simulink model "adrc_main"  (R2025b)
settings: Solver=VariableStepAuto  StartTime=0.0  StopTime=20  RelTol=1e-4
values from neighbouring files (symbols this model uses):
  Alloc = [ kf,     kf,     kf,     kf ... (first row only)    [quad_params.m]
  Area = 2*L*Width    (= 0.072)    [quad_params.m]
  g = 9.81    [quad_params.m]
  h = [0 ... (first row only)    [Madgwick.m]    (also in quad_params.m = 0.2; umich_learning.m = x(:,1))
  h0 = Ts    (= 0.001)    [quad_params.m]
  inertia_mx = [Ixx; Iyy; Izz;]    [quad_params.m]
  init_h = 0.03    [quad_params.m]
  K_alloc = Alloc \ diag([W, 1, 1, 1])    [quad_params.m]
  max_rad_s_2 = max_rad_s ^ 2    (= 4279618.17072)    [quad_params.m]
  max_thrust = max_rad_s_2 * kf * 4    (= 26.9016798211)    [quad_params.m]
  r0_position = 1    [quad_params.m]
  rho_air = 1.225    [quad_params.m]
  rho_water = 1000    [quad_params.m]
  Trot = 0.01    [quad_params.m]
  Ts = 0.001    [get_noise.m]    (also in quad_params.m; test.m = 0.002)
  W = 0.7 + 4*m_prop    (= 0.74)    [quad_params.m]
undefined symbols (not defined in the file or in its folder): adrc
libraries: simulink x4, aerolibwind2 x1
settings Model: PacingRate=0.400000  Creator=David  LastModifiedBy=David

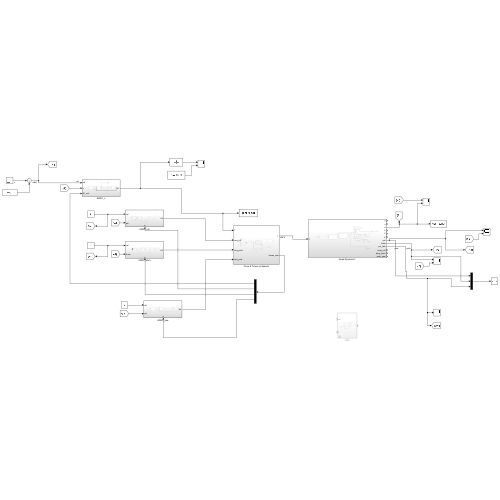
[thumbnail: Simulink's stored preview of the top-level diagram]
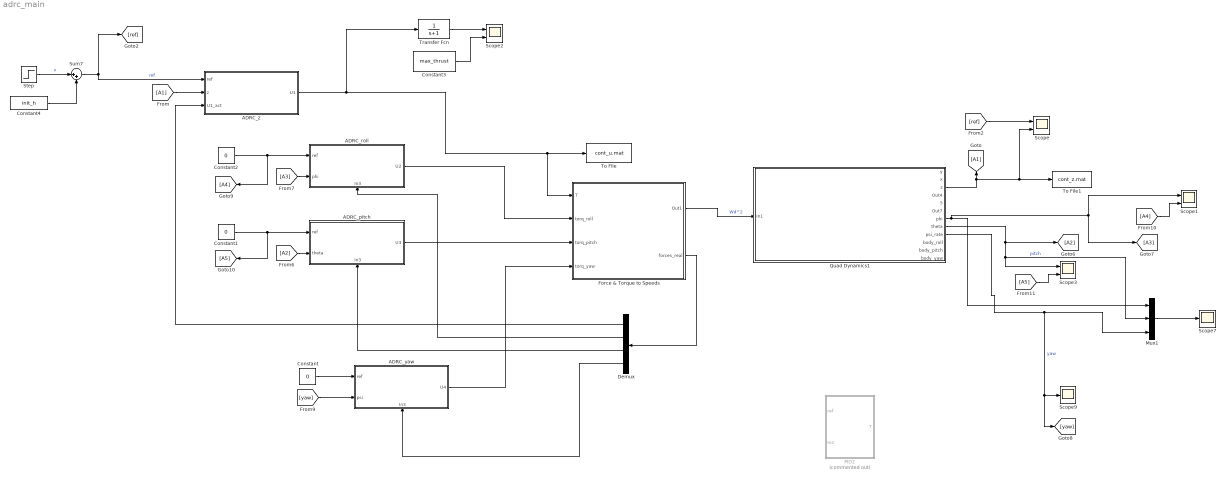
== system adrc_main ==
  ADRC_pitch : Subsystem
      settings: PortSchema="{\"entries\":[{\"content\":{\"sides\":[{\"content\":{\"connectorIds\":[\"In1\",\"In2\"]},\"type\":\"ConnectorPlacement.EquallySpacedRectSide\",\"uuid\":\"6cc80560-d5fb-4d70-bab2-c51ed037dc75\"},{\"content\":{\"connectorIds\":[\"Out1\"],\"side\":\"RIGHT\"},\"type\":\"ConnectorPlacement.EquallySpacedRectSide\",\"uuid\":\"11bda7cd-3ac7-47c0-848b-d0ab204a3c3d\"},{\"content\":{\"side\":\"TOP\"},\"type\":\"ConnectorPlacement.EquallySpacedRectSide\",\"uuid\":\"2a4fd4ae-6a0e-48eb-9f11-b11d2041070f\"},{\"content\":{\"connectorIds\":[\"In3\"],\"side\":\"BOTTOM\"},\"type\":\"ConnectorPlacement.EquallySpacedRectSide\",\"uuid\":\"f4a2dede-c3a4-45a0-96a3-5f68fdbf4ab0\"}]},\"type\":\"ConnectorPlacement.EquallySpacedConnector\",\"uuid\":\"bf44a222-f2d1-4d7f-8b8f-a2aef4aa21c8\"}],\"packageUris\":[\"http://schema.mathworks.com/mf0/Connector/R2020b\"],\"version\":\"1.0\"}"
  ADRC_roll : Subsystem
      settings: PortSchema="{\"entries\":[{\"content\":{\"sides\":[{\"content\":{\"connectorIds\":[\"In1\",\"In2\"]},\"type\":\"ConnectorPlacement.EquallySpacedRectSide\",\"uuid\":\"6cc80560-d5fb-4d70-bab2-c51ed037dc75\"},{\"content\":{\"connectorIds\":[\"Out1\"],\"side\":\"RIGHT\"},\"type\":\"ConnectorPlacement.EquallySpacedRectSide\",\"uuid\":\"11bda7cd-3ac7-47c0-848b-d0ab204a3c3d\"},{\"content\":{\"side\":\"TOP\"},\"type\":\"ConnectorPlacement.EquallySpacedRectSide\",\"uuid\":\"2a4fd4ae-6a0e-48eb-9f11-b11d2041070f\"},{\"content\":{\"connectorIds\":[\"In3\"],\"side\":\"BOTTOM\"},\"type\":\"ConnectorPlacement.EquallySpacedRectSide\",\"uuid\":\"852e14b7-d2e0-4511-9e4e-b55cc1d4afdd\"}]},\"type\":\"ConnectorPlacement.EquallySpacedConnector\",\"uuid\":\"bf44a222-f2d1-4d7f-8b8f-a2aef4aa21c8\"}],\"packageUris\":[\"http://schema.mathworks.com/mf0/Connector/R2020b\"],\"version\":\"1.0\"}"
  ADRC_yaw : Subsystem
      settings: PortSchema="{\"entries\":[{\"content\":{\"sides\":[{\"content\":{\"connectorIds\":[\"In1\",\"In2\"]},\"type\":\"ConnectorPlacement.EquallySpacedRectSide\",\"uuid\":\"6cc80560-d5fb-4d70-bab2-c51ed037dc75\"},{\"content\":{\"connectorIds\":[\"Out1\"],\"side\":\"RIGHT\"},\"type\":\"ConnectorPlacement.EquallySpacedRectSide\",\"uuid\":\"11bda7cd-3ac7-47c0-848b-d0ab204a3c3d\"},{\"content\":{\"side\":\"TOP\"},\"type\":\"ConnectorPlacement.EquallySpacedRectSide\",\"uuid\":\"2a4fd4ae-6a0e-48eb-9f11-b11d2041070f\"},{\"content\":{\"connectorIds\":[\"In3\"],\"side\":\"BOTTOM\"},\"type\":\"ConnectorPlacement.EquallySpacedRectSide\",\"uuid\":\"76ba5801-5866-4633-be25-22afc3afb05e\"}]},\"type\":\"ConnectorPlacement.EquallySpacedConnector\",\"uuid\":\"bf44a222-f2d1-4d7f-8b8f-a2aef4aa21c8\"}],\"packageUris\":[\"http://schema.mathworks.com/mf0/Connector/R2020b\"],\"version\":\"1.0\"}"
  ADRC_z : Subsystem
  Constant : Constant  Value=0
  Constant1 : Constant  Value=0
  Constant2 : Constant  Value=0
  Constant3 : Constant  Value=max_thrust
  Constant4 : Constant  Value=init_h
  Demux : Demux
  Force & Torque to Speeds : Subsystem
  Mux1 : Mux  Inputs=3
  PID2 : Subsystem  Commented=on
  Quad Dynamics1 : Subsystem
  Scope{,1..3} (4 alike) : Scope  NumInputPorts=2
      Scope settings: ActiveDisplayYMinimum=-0.13072157560972555  ActiveDisplayYMaximum=1.1764941804875302  DataLoggingVariableName=ScopeData2
      Scope1 settings: ActiveDisplayYMinimum=-0.066210271925645478  ActiveDisplayYMaximum=0.59589244733080937
      Scope2 settings: ActiveDisplayYMinimum=-1  ActiveDisplayYMaximum=1  DataLoggingVariableName=ScopeData5
      Scope3 settings: ActiveDisplayYMinimum=-0.25349599567622344  ActiveDisplayYMaximum=0.40002228208849239
  Scope7 : Scope
      settings: ActiveDisplayYMinimum=-0.926750348726782  ActiveDisplayYMaximum=1.337695858172476  DataLoggingVariableName=ScopeData16
  Scope9 : Scope
      settings: ActiveDisplayYMinimum=-327.86369595183078  ActiveDisplayYMaximum=1369.6610229277119  DataLoggingVariableName=ScopeData15
  Step : Step  Time=2  SampleTime=0
  Sum7 : Sum  Inputs=|++
  To File : ToFile  Filename=cont_u.mat  SaveFormat=Timeseries
  To File1 : ToFile  Filename=cont_z.mat  SaveFormat=Timeseries
  Transfer Fcn : TransferFcn  Denominator=[1 1]
  wires:
  Quad Dynamics1/3(z) -> To File1/1, Scope/2, [A1]
  [A1] -> ADRC_z/2(z)
  Constant2/1 -> ADRC_roll/1(ref), [A4]
  Constant1/1 -> [A5], ADRC_pitch/1(ref)
  [A2] -> ADRC_pitch/2(theta)
  [A3] -> ADRC_roll/2(phi)
  [yaw] -> ADRC_yaw/2(psi)
  Force & Torque to Speeds/1(Out1) -> Quad Dynamics1/1(In1)  "Wd^2"
  ADRC_z/1(U1) -> Transfer Fcn/1, To File/1, Force & Torque to Speeds/1(T)
  [A4] -> Scope1/2
  [A5] -> Scope3/2
  Quad Dynamics1/9(psi_rate) -> Mux1/3, Scope9/1, [yaw]  "yaw"
  Quad Dynamics1/8(theta) -> [A2], Mux1/2, Scope3/1  "pitch"
  Constant/1 -> ADRC_yaw/1(ref)
  Quad Dynamics1/7(phi) -> Mux1/1, Scope1/1, [A3]
  Force & Torque to Speeds/2(forces_real) -> Demux/1
  Demux/1 -> ADRC_z/3(U1_act)
  Demux/3 -> ADRC_pitch/3(In3)
  Demux/4 -> ADRC_yaw/3(In3)
  Demux/2 -> ADRC_roll/3(In3)
  [ref] -> Scope/1
  Sum7/1 -> [ref], ADRC_z/1(ref)  "ref"
  Step/1 -> Sum7/1  "v"
  Constant4/1 -> Sum7/2
  Mux1/1 -> Scope7/1
  Constant3/1 -> Scope2/2
  Transfer Fcn/1 -> Scope2/1
  ADRC_pitch/1(U3) -> Force & Torque to Speeds/3(torq_pitch)
  ADRC_roll/1(U2) -> Force & Torque to Speeds/2(torq_roll)
  ADRC_yaw/1(U4) -> Force & Torque to Speeds/4(torq_yaw)

== system adrc_main/ADRC_pitch ==
  ref : Inport
  theta : Inport  Port=2
  In3 : Inport  Port=3
  Bus Selector1 : BusSelector  Commented=on  OutputSignals=x3,x1
  LADRC1 : Subsystem
  LESO : Subsystem
  Scope : Scope  NumInputPorts=2
      settings: ActiveDisplayYMinimum=-0.19035360050017919  ActiveDisplayYMaximum=0.29946548587767807  DataLoggingVariableName=ScopeData3
  Scope1 : Scope  NumInputPorts=2
      settings: ActiveDisplayYMinimum=-1.7064424027385405  ActiveDisplayYMaximum=1.5214383476696569  DataLoggingVariableName=ScopeData9
  Scope6 : Scope  Commented=on
      settings: ActiveDisplayYMinimum=-1.7735639903680922  ActiveDisplayYMaximum=2.4901305931130953  DataLoggingVariableName=ScopeData11
  Scope7 : Scope  Commented=on  NumInputPorts=2
      settings: ActiveDisplayYMinimum=-10.826635982413356  ActiveDisplayYMaximum=4.5963077407770285  DataLoggingVariableName=ScopeData7
  Transfer Fcn : TransferFcn  Commented=on  Denominator=[0.8 1]
  Transfer Fcn1 : TransferFcn  Numerator=[1 0]  Denominator=[Ts 1]
  U3 : Outport
  wires:
  Transfer Fcn/1 -> Scope7/2
  ref/1 -> LADRC1/1(ref), Scope/1, Transfer Fcn1/1, Scope/2
  LESO/1(z_hat) -> LADRC1/2(x_hat), Bus Selector1/1
  theta/1 -> LESO/1(theta)
  Bus Selector1/1 -> Transfer Fcn/1, Scope7/1  "<x3>"
  Bus Selector1/2 -> Scope6/1  "<x1>"
  LADRC1/1(U3) -> Scope1/2, U3/1
  Transfer Fcn1/1 -> LADRC1/3(ref_dot)
  In3/1 -> Scope1/1, LESO/2(U3)

== system adrc_main/ADRC_roll ==
  ref : Inport
  phi : Inport  Port=2
  In3 : Inport  Port=3
  Bus Selector1 : BusSelector  Commented=on  OutputSignals=x3,x1
  LADRC1 : Subsystem
  LESO1 : Subsystem
  Scope : Scope  NumInputPorts=2
      settings: ActiveDisplayYMinimum=-0.25662655483048824  ActiveDisplayYMaximum=0.1660137932117976  DataLoggingVariableName=ScopeData25
  Scope1 : Scope  NumInputPorts=2
      settings: ActiveDisplayYMinimum=-1.3986509021572997  ActiveDisplayYMaximum=1.4330939530069289  DataLoggingVariableName=ScopeData14
  Scope6 : Scope  Commented=on
      settings: ActiveDisplayYMinimum=-1.7735639903680922  ActiveDisplayYMaximum=2.4901305931130953  DataLoggingVariableName=ScopeData11
  Scope7 : Scope  Commented=on  NumInputPorts=2
      settings: ActiveDisplayYMinimum=-10.826635982413356  ActiveDisplayYMaximum=4.5963077407770285  DataLoggingVariableName=ScopeData7
  Transfer Fcn : TransferFcn  Commented=on  Denominator=[0.8 1]
  Transfer Fcn1 : TransferFcn  Numerator=[1 0]  Denominator=[Ts 1]
  U2 : Outport
  wires:
  Bus Selector1/2 -> Scope6/1  "<x1>"
  Bus Selector1/1 -> Scope7/1, Transfer Fcn/1  "<x3>"
  phi/1 -> LESO1/1(phi)
  LESO1/1(z_hat) -> LADRC1/2(x_hat)
  Transfer Fcn/1 -> Scope7/2
  Transfer Fcn1/1 -> LADRC1/3(ref_dot)
  ref/1 -> Scope/1, LADRC1/1(ref), Transfer Fcn1/1, Scope/2
  LADRC1/1(U2) -> Scope1/2, U2/1
  In3/1 -> Scope1/1, LESO1/2(U2)

== system adrc_main/ADRC_yaw ==
  ref : Inport
  psi : Inport  Port=2
  In3 : Inport  Port=3
  LADRC1 : Subsystem
  LESO1 : Subsystem
  TD1 : Subsystem
  U4 : Outport
  wires:
  TD1/1(ref) -> LADRC1/1(ref)
  LESO1/1(x_hat) -> LADRC1/2(x_hat)
  psi/1 -> LESO1/1(psi)
  TD1/2(dref) -> LADRC1/3(ref_dot)
  ref/1 -> TD1/1(v)
  In3/1 -> LESO1/2(U4)  "U4_real"
  LADRC1/1(U4) -> U4/1

== system adrc_main/ADRC_z ==
  ref : Inport
  z : Inport  Port=2
  U1_act : Inport  Port=3
  Gain1 : Gain  Gain=1/W
  LADRC1 : Subsystem
  LESO1 : Subsystem
  Scope1 : Scope  NumInputPorts=2
      settings: ActiveDisplayYMinimum=-37.94825498232003  ActiveDisplayYMaximum=51.771622737675379  DataLoggingVariableName=ScopeData21
  TD1 : Subsystem
  U1 : Outport
  wires:
  ref/1 -> TD1/1(v)
  TD1/2(dref) -> LADRC1/3(ref_dot)
  LADRC1/1(U1) -> Scope1/1, Gain1/1
  z/1 -> LESO1/1(z)
  LESO1/1(z_hat) -> LADRC1/2(x_hat)
  TD1/1(ref) -> LADRC1/1(ref)
  Gain1/1 -> U1/1
  U1_act/1 -> LESO1/2(U1), Scope1/2

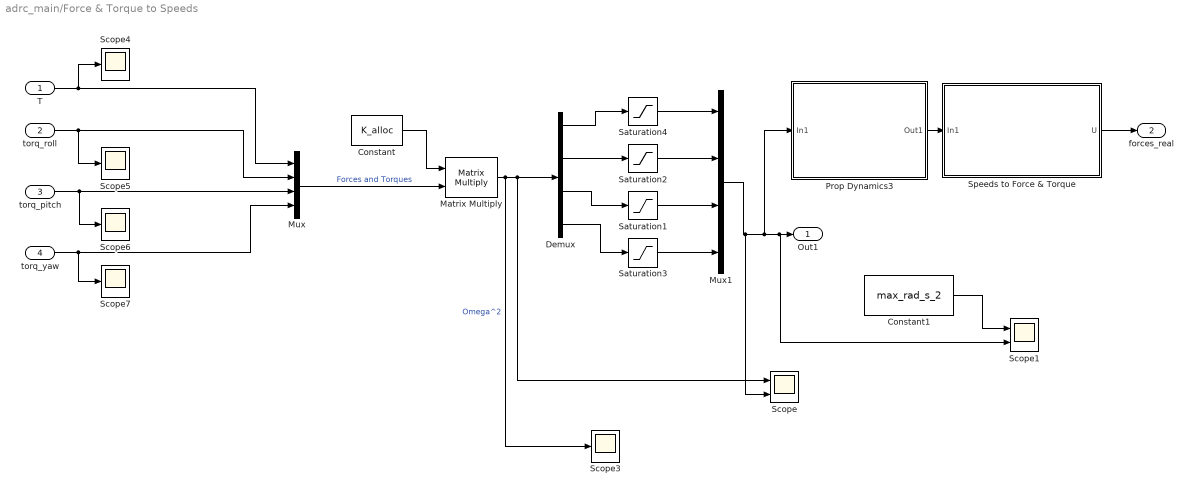
== system adrc_main/Force & Torque to Speeds ==
  T : Inport
  torq_roll : Inport  Port=2
  torq_pitch : Inport  Port=3
  torq_yaw : Inport  Port=4
  Constant : Constant  Value=K_alloc
  Constant1 : Constant  Value=max_rad_s_2
  Demux : Demux
  Matrix Multiply : Product  Multiplication=Matrix(*)
  Mux : Mux
  Mux1 : Mux
  Prop Dynamics3 : Subsystem
  Saturation{1..4} (4 alike) : Saturate  UpperLimit=max_rad_s_2  LowerLimit=0
  Scope : Scope  NumInputPorts=2
      settings: ActiveDisplayYMinimum=-1.1832105851156231E+7  ActiveDisplayYMaximum=1.5311490525694614E+7  DataLoggingVariableName=ScopeData11
  Scope1 : Scope  NumInputPorts=2
      settings: ActiveDisplayYMinimum=-845917.28935251338  ActiveDisplayYMaximum=5.3988813885811847E+6  DataLoggingVariableName=ScopeData25
  Scope{3..7} (5 alike) : Scope
      Scope3 settings: ActiveDisplayYMinimum=-1.1545612320423638E+7  ActiveDisplayYMaximum=1.430543184800574E+7  DataLoggingVariableName=ScopeData24
      Scope4 settings: ActiveDisplayYMinimum=-18.530778781079604  ActiveDisplayYMaximum=17.95290772841328  DataLoggingVariableName=ScopeData27
      Scope5 settings: ActiveDisplayYMinimum=-27.408261850577894  ActiveDisplayYMaximum=37.37109305567089  DataLoggingVariableName=ScopeData28
      Scope6 settings: ActiveDisplayYMinimum=-27.408261850577894  ActiveDisplayYMaximum=37.37109305567089  DataLoggingVariableName=ScopeData29
      Scope7 settings: ActiveDisplayYMinimum=-27.408261850577894  ActiveDisplayYMaximum=37.37109305567089  DataLoggingVariableName=ScopeData30
  Speeds to Force & Torque : Subsystem
  Out1 : Outport
  forces_real : Outport  Port=2
  wires:
  Matrix Multiply/1 -> Scope3/1, Scope/1, Demux/1  "Omega^2"
  torq_yaw/1 -> Mux/4, Scope7/1
  torq_pitch/1 -> Mux/3, Scope6/1
  torq_roll/1 -> Mux/2, Scope5/1
  T/1 -> Mux/1, Scope4/1
  Constant/1 -> Matrix Multiply/1
  Mux/1 -> Matrix Multiply/2  "Forces and Torques"
  Saturation3/1 -> Mux1/4
  Demux/4 -> Saturation3/1
  Demux/2 -> Saturation2/1
  Demux/1 -> Saturation4/1
  Demux/3 -> Saturation1/1
  Saturation2/1 -> Mux1/2
  Saturation4/1 -> Mux1/1
  Saturation1/1 -> Mux1/3
  Mux1/1 -> Scope/2, Scope1/2, Out1/1, Prop Dynamics3/1(In1)
  Speeds to Force & Torque/1(U) -> forces_real/1
  Prop Dynamics3/1(Out1) -> Speeds to Force & Torque/1(In1)
  Constant1/1 -> Scope1/1

== system adrc_main/PID2 ==
  ref : Inport
  In2 : Inport  Port=2
  Gain : Gain  Gain=90
  Gain1 : Gain  Gain=20
  Gain2 : Gain  Gain=30
  Scope : Scope  NumInputPorts=3
      settings: ActiveDisplayYMinimum=-207.05131739453731  ActiveDisplayYMaximum=124.29017503107066  DataLoggingVariableName=ScopeData6
  Sum : Sum  Inputs=|+-
  Sum1 : Sum  Inputs=|+++
  Transfer Fcn : TransferFcn  Numerator=[1 0]  Denominator=[0.01 1]
  Transfer Fcn1 : TransferFcn  Denominator=[1 0]
  T : Outport
  wires:
  In2/1 -> Sum/2
  ref/1 -> Sum/1
  Sum/1 -> Gain2/1, Gain/1, Gain1/1
  Gain1/1 -> Transfer Fcn/1
  Gain2/1 -> Transfer Fcn1/1
  Gain/1 -> Scope/2, Sum1/1  "P"
  Transfer Fcn1/1 -> Sum1/3, Scope/1  "I"
  Transfer Fcn/1 -> Scope/3, Sum1/2  "D"
  Sum1/1 -> T/1

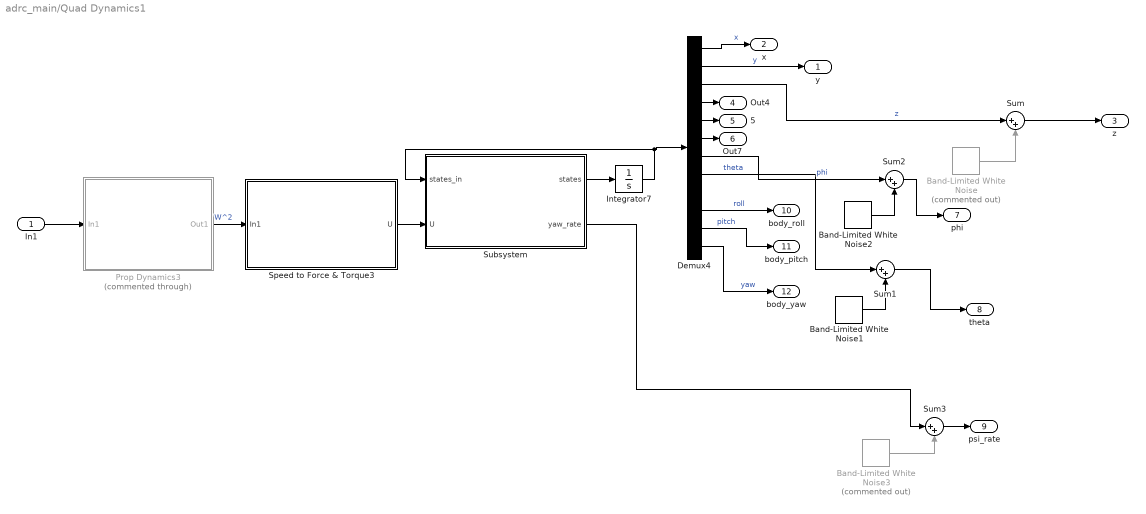
== system adrc_main/Quad Dynamics1 ==
  In1 : Inport
  Band-Limited White Noise : simulink/Sources/Band-Limited White Noise  Commented=on  Cov=[2.6540e-06]  Ts=0.02  seed=[23341]
  Band-Limited White Noise1 : simulink/Sources/Band-Limited White Noise  Cov=[2e-6]  Ts=0.001  seed=[23342]
  Band-Limited White Noise2 : simulink/Sources/Band-Limited White Noise  Cov=[2e-6]  Ts=0.001  seed=[23341]
  Band-Limited White Noise3 : simulink/Sources/Band-Limited White Noise  Commented=on  Cov=[0.0021446]  Ts=0.001  seed=[23343]
  Demux4 : Demux  Outputs=12
  Integrator7 : Integrator  InitialCondition=zeros(12,1)
  Prop Dynamics3 : Subsystem  Commented=through
  Speed to Force & Torque3 : Subsystem
  Subsystem : Subsystem
  Sum{,1..3} (4 alike) : Sum  Inputs=|++
  y : Outport
  x : Outport  Port=2
  z : Outport  Port=3
  Out4 : Outport  Port=4
  5 : Outport  Port=5
  Out7 : Outport  Port=6
  phi : Outport  Port=7
  theta : Outport  Port=8
  psi_rate : Outport  Port=9
  body_roll : Outport  Port=10
  body_pitch : Outport  Port=11
  body_yaw : Outport  Port=12
  wires:
  Demux4/2 -> y/1  "y"
  Prop Dynamics3/1(Out1) -> Speed to Force & Torque3/1(In1)  "W^2"
  Demux4/1 -> x/1  "x"
  Subsystem/1(states) -> Integrator7/1
  Speed to Force & Torque3/1(U) -> Subsystem/2(U)
  Integrator7/1 -> Demux4/1, Subsystem/1(states_in)
  Demux4/10 -> body_roll/1  "roll"
  Demux4/7 -> Sum2/1  "phi"
  Demux4/3 -> Sum/1  "z"
  Demux4/8 -> Sum1/1  "theta"
  Demux4/11 -> body_pitch/1  "pitch"
  Demux4/12 -> body_yaw/1  "yaw"
  Demux4/6 -> Out7/1
  Demux4/5 -> 5/1
  Demux4/4 -> Out4/1
  In1/1 -> Prop Dynamics3/1(In1)
  Subsystem/2(yaw_rate) -> Sum3/1
  Sum/1 -> z/1
  Band-Limited White Noise/1 -> Sum/2
  Band-Limited White Noise1/1 -> Sum1/2
  Sum1/1 -> theta/1
  Band-Limited White Noise2/1 -> Sum2/2
  Sum2/1 -> phi/1
  Band-Limited White Noise3/1 -> Sum3/2
  Sum3/1 -> psi_rate/1

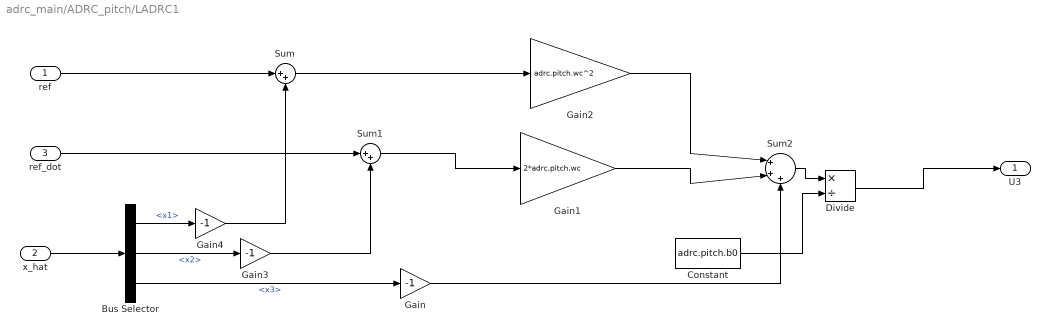
== system adrc_main/ADRC_pitch/LADRC1 ==
  ref : Inport
  x_hat : Inport  Port=2
  ref_dot : Inport  Port=3
  Bus Selector : BusSelector  OutputSignals=x1,x2,x3
  Constant : Constant  Value=adrc.pitch.b0
  Divide : Product  Inputs=*/
  Gain : Gain  Gain=-1
  Gain1 : Gain  Gain=2*adrc.pitch.wc
  Gain2 : Gain  Gain=adrc.pitch.wc^2
  Gain3 : Gain  Gain=-1
  Gain4 : Gain  Gain=-1
  Sum : Sum  Inputs=|++
  Sum1 : Sum  Inputs=|++
  Sum2 : Sum  Inputs=|+++
  U3 : Outport
  wires:
  ref_dot/1 -> Sum1/1
  x_hat/1 -> Bus Selector/1
  Bus Selector/3 -> Gain/1  "<x3>"
  Gain2/1 -> Sum2/1
  Gain/1 -> Sum2/3
  Gain1/1 -> Sum2/2
  Bus Selector/1 -> Gain4/1  "<x1>"
  Bus Selector/2 -> Gain3/1  "<x2>"
  Gain4/1 -> Sum/2
  Gain3/1 -> Sum1/2
  Sum1/1 -> Gain1/1
  Divide/1 -> U3/1
  ref/1 -> Sum/1
  Sum/1 -> Gain2/1
  Sum2/1 -> Divide/1
  Constant/1 -> Divide/2

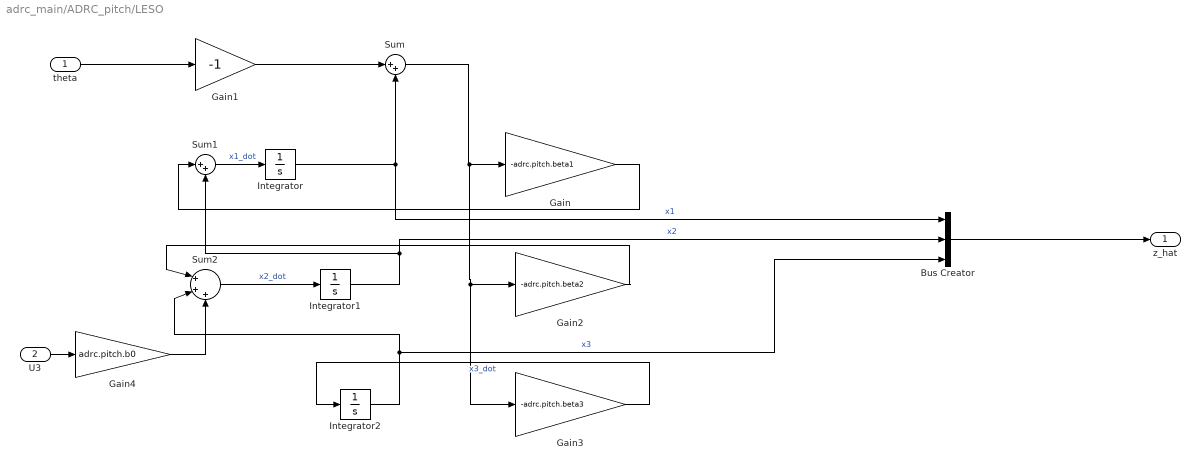
== system adrc_main/ADRC_pitch/LESO ==
  theta : Inport
  U3 : Inport  Port=2
  Bus Creator : BusCreator  Inputs=3
  Gain : Gain  Gain=-adrc.pitch.beta1
  Gain1 : Gain  Gain=-1
  Gain2 : Gain  Gain=-adrc.pitch.beta2
  Gain3 : Gain  Gain=-adrc.pitch.beta3
  Gain4 : Gain  Gain=adrc.pitch.b0
  Integrator : Integrator
  Integrator1 : Integrator
  Integrator2 : Integrator
  Sum : Sum  Inputs=|++
  Sum1 : Sum  Inputs=|++
  Sum2 : Sum  Inputs=|+++
  z_hat : Outport
  wires:
  theta/1 -> Gain1/1
  Gain1/1 -> Sum/1
  Sum/1 -> Gain3/1, Gain2/1, Gain/1
  Integrator/1 -> Bus Creator/1, Sum/2  "x1"
  Gain3/1 -> Integrator2/1  "x3_dot"
  Bus Creator/1 -> z_hat/1
  Sum1/1 -> Integrator/1  "x1_dot"
  Gain/1 -> Sum1/1
  Integrator1/1 -> Bus Creator/2, Sum1/2  "x2"
  Integrator2/1 -> Bus Creator/3, Sum2/2  "x3"
  Gain2/1 -> Sum2/1
  Sum2/1 -> Integrator1/1  "x2_dot"
  U3/1 -> Gain4/1
  Gain4/1 -> Sum2/3

== system adrc_main/ADRC_roll/LADRC1 ==
  ref : Inport
  x_hat : Inport  Port=2
  ref_dot : Inport  Port=3
  Bus Selector : BusSelector  OutputSignals=x1,x2,x3
  Constant : Constant  Value=adrc.roll.b0
  Divide : Product  Inputs=*/
  Gain : Gain  Gain=-1
  Gain1 : Gain  Gain=2*adrc.roll.wc
  Gain2 : Gain  Gain=adrc.roll.wc^2
  Gain3 : Gain  Gain=-1
  Gain4 : Gain  Gain=-1
  Sum : Sum  Inputs=|++
  Sum1 : Sum  Inputs=|++
  Sum2 : Sum  Inputs=|+++
  U2 : Outport
  wires:
  ref_dot/1 -> Sum1/1
  x_hat/1 -> Bus Selector/1
  Bus Selector/3 -> Gain/1  "<x3>"
  Gain2/1 -> Sum2/1
  Gain/1 -> Sum2/3
  Gain1/1 -> Sum2/2
  Bus Selector/1 -> Gain4/1  "<x1>"
  Bus Selector/2 -> Gain3/1  "<x2>"
  Gain4/1 -> Sum/2
  Gain3/1 -> Sum1/2
  Sum1/1 -> Gain1/1
  Divide/1 -> U2/1
  ref/1 -> Sum/1
  Sum/1 -> Gain2/1
  Sum2/1 -> Divide/1
  Constant/1 -> Divide/2

== system adrc_main/ADRC_roll/LESO1 ==
  phi : Inport
  U2 : Inport  Port=2
  Bus Creator : BusCreator  Inputs=3
  Gain : Gain  Gain=-adrc.roll.beta1
  Gain1 : Gain  Gain=-1
  Gain2 : Gain  Gain=-adrc.roll.beta2
  Gain3 : Gain  Gain=-adrc.roll.beta3
  Gain4 : Gain  Gain=adrc.roll.b0
  Integrator : Integrator
  Integrator1 : Integrator
  Integrator2 : Integrator
  Sum : Sum  Inputs=|++
  Sum1 : Sum  Inputs=|++
  Sum2 : Sum  Inputs=|+++
  z_hat : Outport
  wires:
  Gain4/1 -> Sum2/3
  U2/1 -> Gain4/1
  Sum2/1 -> Integrator1/1  "x2_dot"
  Gain2/1 -> Sum2/1
  Integrator2/1 -> Sum2/2, Bus Creator/3  "x3"
  Integrator1/1 -> Sum1/2, Bus Creator/2  "x2"
  Gain/1 -> Sum1/1
  Sum1/1 -> Integrator/1  "x1_dot"
  Bus Creator/1 -> z_hat/1
  Gain3/1 -> Integrator2/1  "x3_dot"
  Integrator/1 -> Sum/2, Bus Creator/1  "x1"
  Sum/1 -> Gain/1, Gain3/1, Gain2/1
  Gain1/1 -> Sum/1
  phi/1 -> Gain1/1

== system adrc_main/ADRC_yaw/LADRC1 ==
  ref : Inport
  x_hat : Inport  Port=2
  ref_dot : Inport  Port=3
  Bus Selector : BusSelector  OutputSignals=x1,x2,x3
  Constant : Constant  Value=adrc.yaw.b0
  Divide : Product  Inputs=*/
  Gain : Gain  Gain=-1
  Gain1 : Gain  Gain=2*adrc.yaw.wc
  Gain2 : Gain  Gain=adrc.yaw.wc^2
  Gain3 : Gain  Gain=-1
  Gain4 : Gain  Gain=-1
  Sum : Sum  Inputs=|++
  Sum1 : Sum  Inputs=|++
  Sum2 : Sum  Inputs=|+++
  U4 : Outport
  wires:
  Sum/1 -> Gain2/1
  ref/1 -> Sum/1
  Sum1/1 -> Gain1/1
  Gain3/1 -> Sum1/2
  Gain4/1 -> Sum/2
  Bus Selector/2 -> Gain3/1  "<x2>"
  Bus Selector/1 -> Gain4/1  "<x1>"
  Gain1/1 -> Sum2/2
  Gain/1 -> Sum2/3
  Gain2/1 -> Sum2/1
  Bus Selector/3 -> Gain/1  "<x3>"
  x_hat/1 -> Bus Selector/1
  Divide/1 -> U4/1
  ref_dot/1 -> Sum1/1
  Sum2/1 -> Divide/1
  Constant/1 -> Divide/2

== system adrc_main/ADRC_yaw/LESO1 ==
  psi : Inport
  U4 : Inport  Port=2
  Bus Creator : BusCreator  Inputs=3
  Gain : Gain  Gain=-adrc.yaw.beta1
  Gain1 : Gain  Gain=-1
  Gain2 : Gain  Gain=-adrc.yaw.beta2
  Gain3 : Gain  Gain=-adrc.yaw.beta3
  Gain4 : Gain  Gain=adrc.yaw.b0
  Integrator : Integrator
  Integrator1 : Integrator
  Integrator2 : Integrator
  Sum : Sum  Inputs=|++
  Sum1 : Sum  Inputs=|++
  Sum2 : Sum  Inputs=|+++
  x_hat : Outport
  wires:
  psi/1 -> Gain1/1
  Gain1/1 -> Sum/1
  Sum/1 -> Gain3/1, Gain2/1, Gain/1
  Integrator/1 -> Bus Creator/1, Sum/2  "x1"
  Gain3/1 -> Integrator2/1  "x3_dot"
  Bus Creator/1 -> x_hat/1
  Sum1/1 -> Integrator/1  "x1_dot"
  Gain/1 -> Sum1/1
  Integrator1/1 -> Bus Creator/2, Sum1/2  "x2"
  Integrator2/1 -> Bus Creator/3, Sum2/2  "x3"
  Gain2/1 -> Sum2/1
  Sum2/1 -> Integrator1/1  "x2_dot"
  U4/1 -> Gain4/1
  Gain4/1 -> Sum2/3

== system adrc_main/ADRC_yaw/TD1 ==
  v : Inport
  Constant11 : Constant  Value=r0_position
  Constant12 : Constant  Value=h0
  Delay One Step : Delay  DelayLength=1  SampleTime=Ts
  Delay One Step1 : Delay  DelayLength=1  SampleTime=Ts
  Gain3 : Gain  Gain=Ts
  Gain4 : Gain  Gain=Ts
  Sum1 : Sum  Inputs=|++
  Sum6 : Sum  Inputs=|++
  Sum7 : Sum  Inputs=|+-
  fhan : MATLAB Function  TreatAsAtomicUnit=on
  ref : Outport
  dref : Outport  Port=2
  wires:
  v/1 -> Sum7/2
  Constant12/1 -> fhan/4(h0)
  Sum7/1 -> fhan/1(e)
  Constant11/1 -> fhan/3(r0)
  Delay One Step1/1 -> fhan/2(v2), Sum6/2, dref/1, Gain4/1  "v2(k)"
  Gain4/1 -> Sum1/2
  Sum1/1 -> Delay One Step/1  "v1(k+1)"
  Sum6/1 -> Delay One Step1/1  "v2(k+1)"
  Gain3/1 -> Sum6/1
  Delay One Step/1 -> ref/1, Sum1/1, Sum7/1  "v1"
  fhan/1(u) -> Gain3/1

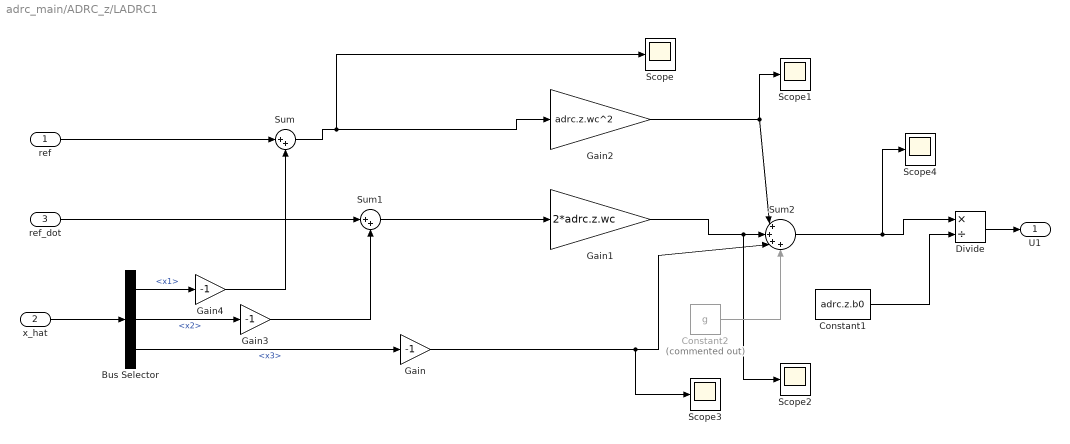
== system adrc_main/ADRC_z/LADRC1 ==
  ref : Inport
  x_hat : Inport  Port=2
  ref_dot : Inport  Port=3
  Bus Selector : BusSelector  OutputSignals=x1,x2,x3
  Constant1 : Constant  Value=adrc.z.b0
  Constant2 : Constant  Commented=on  Value=g
  Divide : Product  Inputs=*/
  Gain : Gain  Gain=-1
  Gain1 : Gain  Gain=2*adrc.z.wc
  Gain2 : Gain  Gain=adrc.z.wc^2
  Gain3 : Gain  Gain=-1
  Gain4 : Gain  Gain=-1
  Scope{,1..4} (5 alike) : Scope
      Scope settings: ActiveDisplayYMinimum=-1  ActiveDisplayYMaximum=1  DataLoggingVariableName=ScopeData13
      Scope1 settings: ActiveDisplayYMinimum=-1  ActiveDisplayYMaximum=1  DataLoggingVariableName=ScopeData17
      Scope2 settings: ActiveDisplayYMinimum=-1  ActiveDisplayYMaximum=1  DataLoggingVariableName=ScopeData18
      Scope3 settings: ActiveDisplayYMinimum=-1  ActiveDisplayYMaximum=1  DataLoggingVariableName=ScopeData19
      Scope4 settings: ActiveDisplayYMinimum=-24.496239741805212  ActiveDisplayYMaximum=21.725148286709803  DataLoggingVariableName=ScopeData20
  Sum : Sum  Inputs=|++
  Sum1 : Sum  Inputs=|++
  Sum2 : Sum  Inputs=|++++
  U1 : Outport
  wires:
  ref_dot/1 -> Sum1/1
  x_hat/1 -> Bus Selector/1
  Bus Selector/3 -> Gain/1  "<x3>"
  Gain2/1 -> Sum2/1, Scope1/1
  Gain/1 -> Scope3/1, Sum2/3
  Gain1/1 -> Scope2/1, Sum2/2
  Bus Selector/1 -> Gain4/1  "<x1>"
  Bus Selector/2 -> Gain3/1  "<x2>"
  Gain4/1 -> Sum/2
  Gain3/1 -> Sum1/2
  Sum1/1 -> Gain1/1
  Divide/1 -> U1/1
  Constant1/1 -> Divide/2
  ref/1 -> Sum/1
  Sum/1 -> Scope/1, Gain2/1
  Sum2/1 -> Scope4/1, Divide/1
  Constant2/1 -> Sum2/4

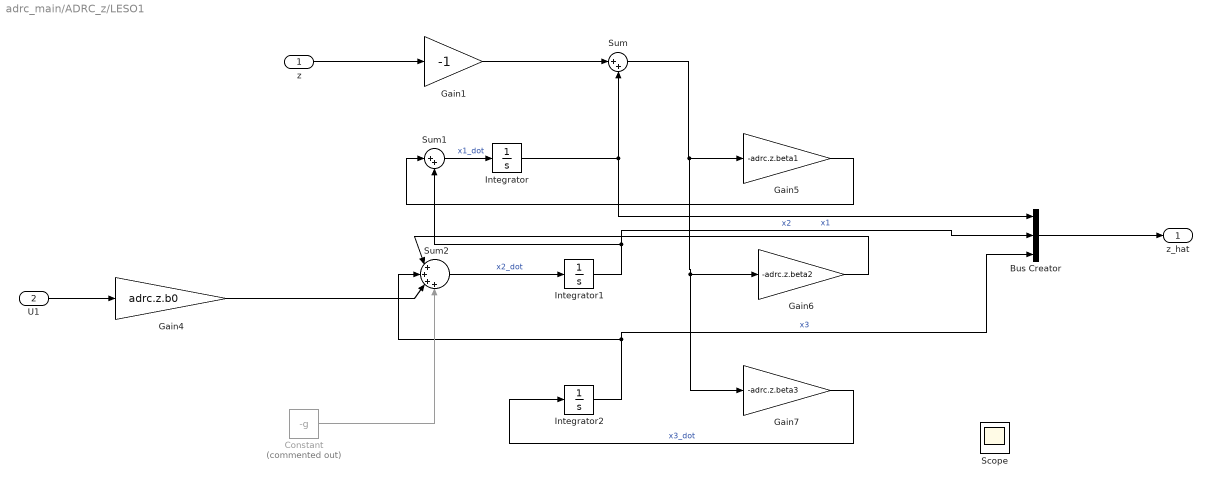
== system adrc_main/ADRC_z/LESO1 ==
  z : Inport
  U1 : Inport  Port=2
  Bus Creator : BusCreator  Inputs=3
  Constant : Constant  Commented=on  Value=-g
  Gain1 : Gain  Gain=-1
  Gain4 : Gain  Gain=adrc.z.b0
  Gain5 : Gain  Gain=-adrc.z.beta1
  Gain6 : Gain  Gain=-adrc.z.beta2
  Gain7 : Gain  Gain=-adrc.z.beta3
  Integrator : Integrator
  Integrator1 : Integrator
  Integrator2 : Integrator
  Scope : Scope
      settings: DataLoggingVariableName=ScopeData12
  Sum : Sum  Inputs=|++
  Sum1 : Sum  Inputs=|++
  Sum2 : Sum  Inputs=|++++
  z_hat : Outport
  wires:
  U1/1 -> Gain4/1
  Sum2/1 -> Integrator1/1  "x2_dot"
  Gain6/1 -> Sum2/1
  Integrator2/1 -> Sum2/2, Bus Creator/3  "x3"
  Integrator1/1 -> Sum1/2, Bus Creator/2  "x2"
  Gain5/1 -> Sum1/1
  Sum1/1 -> Integrator/1  "x1_dot"
  Bus Creator/1 -> z_hat/1
  Gain7/1 -> Integrator2/1  "x3_dot"
  Integrator/1 -> Sum/2, Bus Creator/1  "x1"
  Sum/1 -> Gain5/1, Gain7/1, Gain6/1
  Gain1/1 -> Sum/1
  z/1 -> Gain1/1
  Constant/1 -> Sum2/4
  Gain4/1 -> Sum2/3

== system adrc_main/ADRC_z/TD1 ==
  v : Inport
  Constant11 : Constant  Value=r0_position
  Constant12 : Constant  Value=h0
  Delay One Step : Delay  DelayLength=1  SampleTime=Ts
  Delay One Step1 : Delay  DelayLength=1  SampleTime=Ts
  Gain3 : Gain  Gain=Ts
  Gain4 : Gain  Gain=Ts
  Sum1 : Sum  Inputs=|++
  Sum6 : Sum  Inputs=|++
  Sum7 : Sum  Inputs=|+-
  fhan : MATLAB Function  TreatAsAtomicUnit=on
  ref : Outport
  dref : Outport  Port=2
  wires:
  v/1 -> Sum7/2
  Constant12/1 -> fhan/4(h0)
  Sum7/1 -> fhan/1(e)
  Constant11/1 -> fhan/3(r0)
  Delay One Step1/1 -> fhan/2(v2), Sum6/2, Gain4/1  "v2(k)"
  Gain4/1 -> Sum1/2
  Sum1/1 -> ref/1, Delay One Step/1  "v1(k+1)"
  Sum6/1 -> dref/1, Delay One Step1/1  "v2(k+1)"
  Gain3/1 -> Sum6/1
  Delay One Step/1 -> Sum1/1, Sum7/1  "v1"
  fhan/1(u) -> Gain3/1

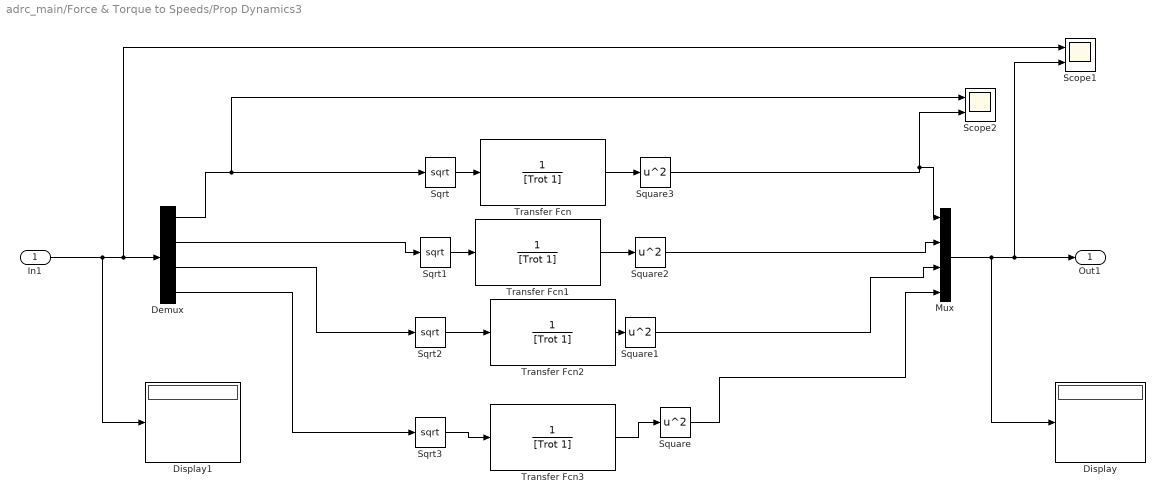
== system adrc_main/Force & Torque to Speeds/Prop Dynamics3 ==
  In1 : Inport
  Demux : Demux
  Display : Display
  Display1 : Display
  Mux : Mux
  Scope1 : Scope  NumInputPorts=2
      settings: ActiveDisplayYMinimum=-1.6200330151208001E+6  ActiveDisplayYMaximum=1.4580297136087205E+7  DataLoggingVariableName=ScopeData22
  Scope2 : Scope  NumInputPorts=2
      settings: ActiveDisplayYMinimum=-993371.3028758571  ActiveDisplayYMaximum=8.9403417258827165E+6  DataLoggingVariableName=ScopeData26
  Sqrt{,1..3} (4 alike) : Sqrt
  Square{,1..3} (4 alike) : Math  Operator=square
  Transfer Fcn{,1..3} (4 alike) : TransferFcn  Denominator=[Trot 1]
  Out1 : Outport
  wires:
  Square/1 -> Mux/4
  Demux/4 -> Sqrt3/1
  Demux/3 -> Sqrt2/1
  Demux/2 -> Sqrt1/1
  Demux/1 -> Sqrt/1, Scope2/1
  Sqrt3/1 -> Transfer Fcn3/1
  Sqrt2/1 -> Transfer Fcn2/1
  Sqrt1/1 -> Transfer Fcn1/1
  Sqrt/1 -> Transfer Fcn/1
  Transfer Fcn3/1 -> Square/1
  Transfer Fcn2/1 -> Square1/1
  Transfer Fcn/1 -> Square3/1
  Transfer Fcn1/1 -> Square2/1
  Mux/1 -> Scope1/2, Out1/1, Display/1
  In1/1 -> Scope1/1, Demux/1, Display1/1
  Square3/1 -> Scope2/2, Mux/1
  Square2/1 -> Mux/2
  Square1/1 -> Mux/3

== system adrc_main/Force & Torque to Speeds/Speeds to Force & Torque ==
  In1 : Inport
  Constant1 : Constant  Value=Alloc
  Matrix Multiply1 : Product  Multiplication=Matrix(*)
  U : Outport
  wires:
  Constant1/1 -> Matrix Multiply1/1
  Matrix Multiply1/1 -> U/1
  In1/1 -> Matrix Multiply1/2  "Omega^2"

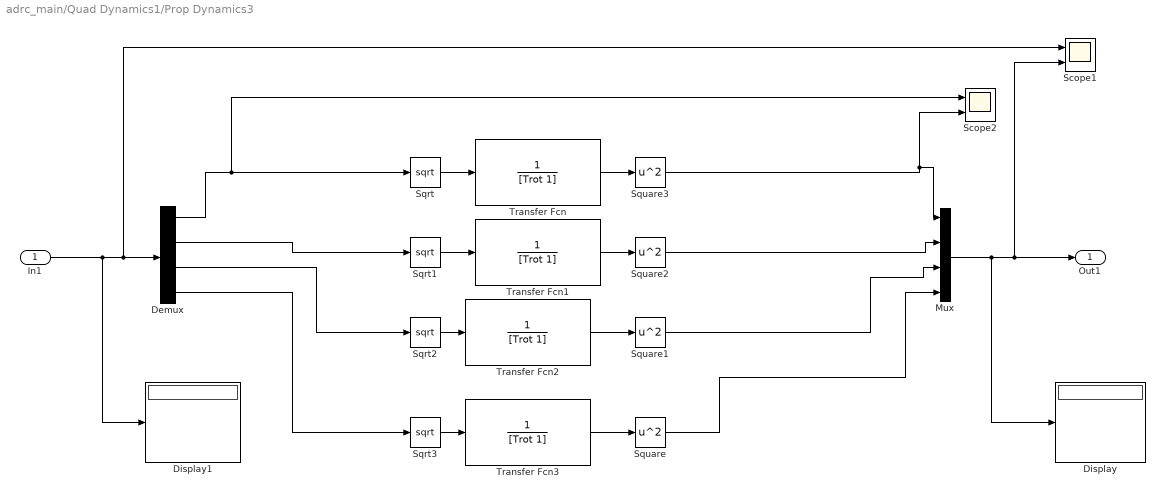
== system adrc_main/Quad Dynamics1/Prop Dynamics3 ==
  In1 : Inport
  Demux : Demux
  Display : Display
  Display1 : Display
  Mux : Mux
  Scope1 : Scope  NumInputPorts=2
      settings: ActiveDisplayYMinimum=-75977.2512965213  ActiveDisplayYMaximum=683795.26166869176  DataLoggingVariableName=ScopeData22
  Scope2 : Scope  NumInputPorts=2
      settings: ActiveDisplayYMinimum=-993371.3028758571  ActiveDisplayYMaximum=8.9403417258827165E+6  DataLoggingVariableName=ScopeData26
  Sqrt{,1..3} (4 alike) : Sqrt
  Square{,1..3} (4 alike) : Math  Operator=square
  Transfer Fcn{,1..3} (4 alike) : TransferFcn  Denominator=[Trot 1]
  Out1 : Outport
  wires:
  Square/1 -> Mux/4
  Demux/4 -> Sqrt3/1
  Demux/3 -> Sqrt2/1
  Demux/2 -> Sqrt1/1
  Demux/1 -> Sqrt/1, Scope2/1
  Sqrt3/1 -> Transfer Fcn3/1
  Sqrt2/1 -> Transfer Fcn2/1
  Sqrt1/1 -> Transfer Fcn1/1
  Sqrt/1 -> Transfer Fcn/1
  Transfer Fcn3/1 -> Square/1
  Transfer Fcn2/1 -> Square1/1
  Transfer Fcn/1 -> Square3/1
  Transfer Fcn1/1 -> Square2/1
  Mux/1 -> Scope1/2, Out1/1, Display/1
  In1/1 -> Scope1/1, Demux/1, Display1/1
  Square3/1 -> Scope2/2, Mux/1
  Square2/1 -> Mux/2
  Square1/1 -> Mux/3

== system adrc_main/Quad Dynamics1/Speed to Force & Torque3 ==
  In1 : Inport
  Constant1 : Constant  Value=Alloc
  Matrix Multiply1 : Product  Multiplication=Matrix(*)
  U : Outport
  wires:
  Constant1/1 -> Matrix Multiply1/1
  Matrix Multiply1/1 -> U/1
  In1/1 -> Matrix Multiply1/2  "Omega^2"

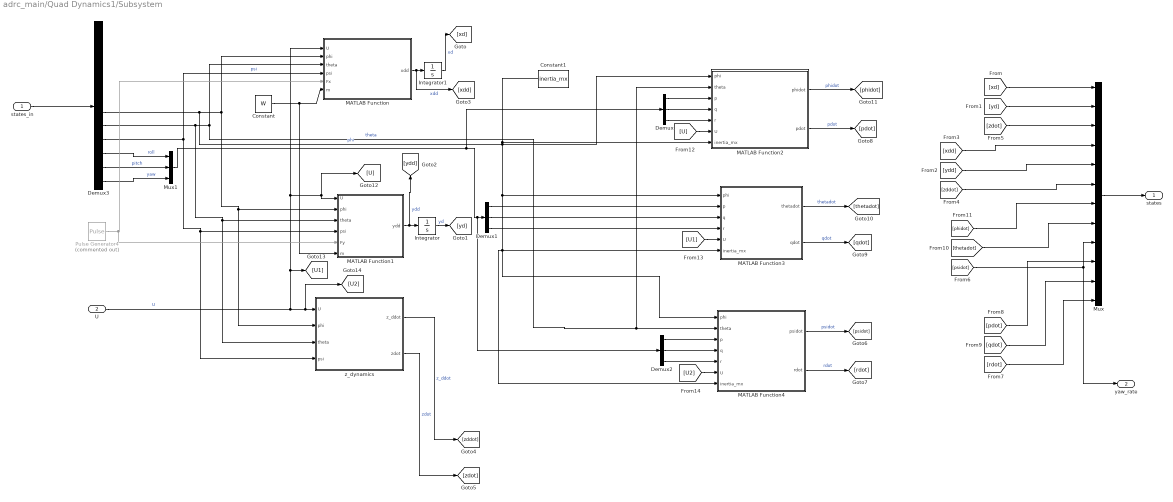
== system adrc_main/Quad Dynamics1/Subsystem ==
  states_in : Inport
  U : Inport  Port=2
  Constant : Constant  Value=W
  Constant1 : Constant  Value=inertia_mx
  Demux : Demux  Outputs=3
  Demux1 : Demux  Outputs=3
  Demux2 : Demux  Outputs=3
  Demux3 : Demux  Outputs=12
  Integrator : Integrator
  Integrator1 : Integrator
  MATLAB Function : MATLAB Function  TreatAsAtomicUnit=on
  MATLAB Function1 : MATLAB Function  TreatAsAtomicUnit=on
  MATLAB Function2 : MATLAB Function  TreatAsAtomicUnit=on
  MATLAB Function3 : MATLAB Function  TreatAsAtomicUnit=on
  MATLAB Function4 : MATLAB Function  TreatAsAtomicUnit=on
  Mux : Mux  Inputs=12
  Mux1 : Mux  Inputs=3
  Pulse Generator4 : DiscretePulseGenerator  Commented=on  PulseType=Time based  Amplitude=0.1  Period=5  PulseWidth=30  PhaseDelay=6
  z_dynamics : Subsystem
  states : Outport
  yaw_rate : Outport  Port=2
  wires:
  MATLAB Function/1(xdd) -> [xdd], Integrator1/1  "xdd"
  MATLAB Function1/1(ydd) -> [ydd], Integrator/1  "ydd"
  Mux/1 -> states/1
  states_in/1 -> Demux3/1
  U/1 -> [U2], z_dynamics/1(U), MATLAB Function/1(U), [U], MATLAB Function1/1(U), [U1]  "U"
  Demux3/7 -> MATLAB Function3/1(phi), MATLAB Function4/1(phi), MATLAB Function2/1(phi), MATLAB Function/2(phi), z_dynamics/2(phi), MATLAB Function1/2(phi)  "phi"
  Demux3/8 -> z_dynamics/3(theta), MATLAB Function1/3(theta), MATLAB Function2/2(theta), MATLAB Function4/2(theta), MATLAB Function/3(theta)  "theta"
  Demux3/9 -> z_dynamics/4(psi), MATLAB Function1/4(psi), MATLAB Function/4(psi)  "psi"
  Constant/1 -> MATLAB Function/6(m), MATLAB Function1/6(m)
  Constant1/1 -> MATLAB Function4/7(inertia_mx), MATLAB Function3/6(inertia_mx), MATLAB Function2/7(inertia_mx)
  Demux3/11 -> Mux1/2  "pitch"
  Demux3/12 -> Mux1/3  "yaw"
  Demux3/10 -> Mux1/1  "roll"
  Mux1/1 -> Demux/1, Demux2/1, Demux1/1
  Demux1/1 -> MATLAB Function3/2(p)
  Demux1/2 -> MATLAB Function3/3(q)
  Demux1/3 -> MATLAB Function3/4(r)
  Demux2/1 -> MATLAB Function4/3(p)
  Demux2/2 -> MATLAB Function4/4(q)
  Demux2/3 -> MATLAB Function4/5(r)
  Demux/1 -> MATLAB Function2/3(p)
  Demux/2 -> MATLAB Function2/4(q)
  Demux/3 -> MATLAB Function2/5(r)
  Integrator1/1 -> [xd]  "xd"
  [xd] -> Mux/1
  Integrator/1 -> [yd]  "yd"
  [yd] -> Mux/2
  [ydd] -> Mux/5
  [xdd] -> Mux/4
  z_dynamics/1(z_ddot) -> [zddot]  "z_ddot"
  [zddot] -> Mux/6
  z_dynamics/2(zdot) -> [zdot]  "zdot"
  [zdot] -> Mux/3
  MATLAB Function4/1(psidot) -> [psidot]  "psidot"
  [psidot] -> Mux/9, yaw_rate/1
  MATLAB Function4/2(rdot) -> [rdot]  "rdot"
  [rdot] -> Mux/12
  MATLAB Function2/2(pdot) -> [pdot]  "pdot"
  [pdot] -> Mux/10
  MATLAB Function3/2(qdot) -> [qdot]  "qdot"
  [qdot] -> Mux/11
  MATLAB Function3/1(thetadot) -> [thetadot]  "thetadot"
  [thetadot] -> Mux/8
  MATLAB Function2/1(phidot) -> [phidot]  "phidot"
  [phidot] -> Mux/7
  [U] -> MATLAB Function2/6(U)
  [U1] -> MATLAB Function3/5(U)
  [U2] -> MATLAB Function4/6(U)
  Pulse Generator4/1 -> MATLAB Function1/5(Fy), MATLAB Function/5(Fx)

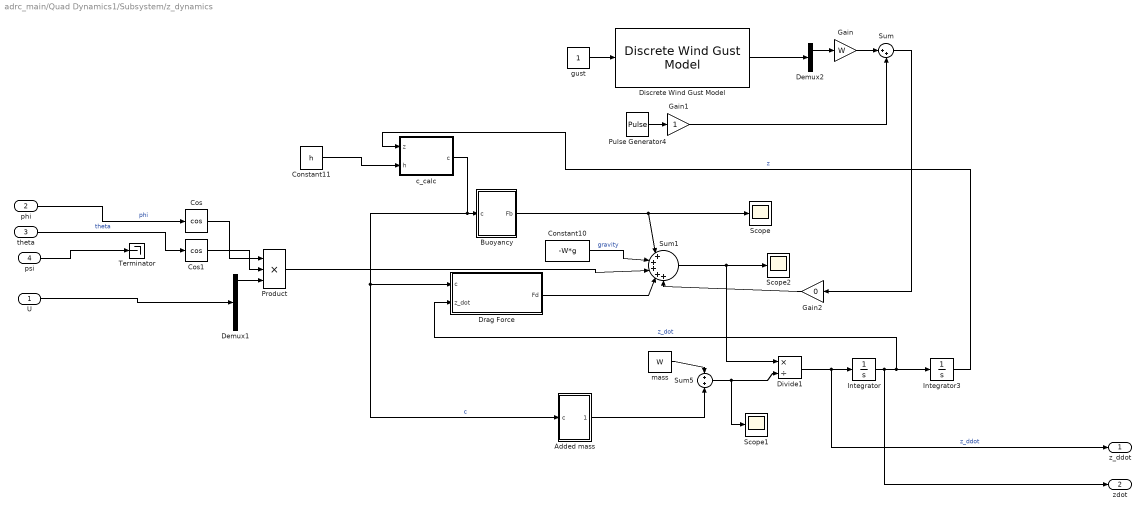
== system adrc_main/Quad Dynamics1/Subsystem/z_dynamics ==
  U : Inport
  phi : Inport  Port=2
  theta : Inport  Port=3
  psi : Inport  Port=4
  Added mass : Subsystem
  Buoyancy : Subsystem
  Constant10 : Constant  Value=-W*g
  Constant11 : Constant  Value=h
  Cos : Trigonometry  Operator=cos
  Cos1 : Trigonometry  Operator=cos
  Demux1 : Demux
  Demux2 : Demux  Outputs=3
  Discrete Wind Gust Model : aerolibwind2/Discrete Wind Gust Model  units=Metric (MKS)  Gx=on  Gy=off  Gz=off  t_0=7  d_m=[1 0.5 0.5]  v_m=[2 2 2]
  Divide1 : Product  Inputs=*/
  Drag Force : Subsystem
  Gain : Gain  Gain=W
  Gain1 : Gain
  Gain2 : Gain  Gain=0
  Integrator : Integrator
  Integrator3 : Integrator
  Product : Product  Inputs=3
  Pulse Generator4 : DiscretePulseGenerator  PulseType=Time based  Amplitude=5  Period=5  PulseWidth=30  PhaseDelay=5
  Scope : Scope
      settings: ActiveDisplayYMinimum=3.324205069659222  ActiveDisplayYMaximum=24.046643881148977  DataLoggingVariableName=ScopeData4
  Scope1 : Scope
      settings: ActiveDisplayYMinimum=1.2962500000000001  ActiveDisplayYMaximum=1.7337500000000001  DataLoggingVariableName=ScopeData8
  Scope2 : Scope
      settings: ActiveDisplayYMinimum=-2.7468  ActiveDisplayYMaximum=24.721200000000003  DataLoggingVariableName=ScopeData10
  Sum : Sum  Inputs=|++
  Sum1 : Sum  Inputs=|+++++
  Sum5 : Sum
  Terminator : Terminator
  c_calc : MATLAB Function  TreatAsAtomicUnit=on
  gust : Constant
  mass : Constant  Value=W
  z_ddot : Outport
  zdot : Outport  Port=2
  wires:
  phi/1 -> Cos/1  "phi"
  theta/1 -> Cos1/1  "theta"
  Cos/1 -> Product/1
  Cos1/1 -> Product/2
  Demux1/1 -> Product/3
  psi/1 -> Terminator/1
  Sum1/1 -> Scope2/1, Divide1/1
  c_calc/1(c) -> Added mass/1(c), Drag Force/1(c), Buoyancy/1(c)  "c"
  Product/1 -> Sum1/3
  Added mass/1(m_a) -> Sum5/2
  mass/1 -> Sum5/1
  Sum5/1 -> Scope1/1, Divide1/2
  Integrator3/1 -> c_calc/1(z)  "z"
  Integrator/1 -> Drag Force/2(z_dot), Integrator3/1, zdot/1  "z_dot"
  Drag Force/1(Fd) -> Sum1/4
  Divide1/1 -> z_ddot/1, Integrator/1  "z_ddot"
  Buoyancy/1(Fb) -> Sum1/1, Scope/1
  Constant10/1 -> Sum1/2  "gravity"
  Constant11/1 -> c_calc/2(h)
  U/1 -> Demux1/1
  Gain1/1 -> Sum/2
  Discrete Wind Gust Model/1 -> Demux2/1
  Demux2/1 -> Gain/1
  Gain/1 -> Sum/1
  Pulse Generator4/1 -> Gain1/1
  Sum/1 -> Gain2/1
  gust/1 -> Discrete Wind Gust Model/1
  Gain2/1 -> Sum1/5

== system adrc_main/Quad Dynamics1/Subsystem/z_dynamics/Added mass ==
  c : Inport
  Product1 : Product
  added_mass : Constant  Value=0.05*rho_water
  m_a : Outport
  wires:
  added_mass/1 -> Product1/1
  Product1/1 -> m_a/1
  c/1 -> Product1/2

== system adrc_main/Quad Dynamics1/Subsystem/z_dynamics/Buoyancy ==
  c : Inport
  Constant1 : Constant  Value=rho_water*Area*g
  Product : Product
  Fb : Outport
  wires:
  Constant1/1 -> Product/2
  c/1 -> Product/1
  Product/1 -> Fb/1  "buoyancy"

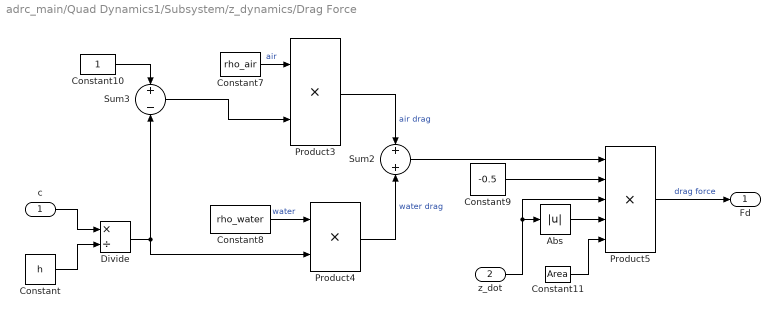
== system adrc_main/Quad Dynamics1/Subsystem/z_dynamics/Drag Force ==
  c : Inport
  z_dot : Inport  Port=2
  Abs : Abs  SaturateOnIntegerOverflow=off
  Constant : Constant  Value=h
  Constant10 : Constant
  Constant11 : Constant  Value=Area
  Constant7 : Constant  Value=rho_air
  Constant8 : Constant  Value=rho_water
  Constant9 : Constant  Value=-0.5
  Divide : Product  Inputs=*/
  Product3 : Product
  Product4 : Product
  Product5 : Product  Inputs=5
  Sum2 : Sum
  Sum3 : Sum  Inputs=+-
  Fd : Outport
  wires:
  Divide/1 -> Sum3/2, Product4/2
  Product5/1 -> Fd/1  "drag force"
  Product4/1 -> Sum2/2  "water drag"
  Constant11/1 -> Product5/5
  Sum3/1 -> Product3/2
  Constant8/1 -> Product4/1  "water"
  Constant10/1 -> Sum3/1
  Sum2/1 -> Product5/1
  Constant9/1 -> Product5/2
  z_dot/1 -> Abs/1, Product5/3
  Abs/1 -> Product5/4
  Product3/1 -> Sum2/1  "air drag"
  Constant7/1 -> Product3/1  "air"
  c/1 -> Divide/1
  Constant/1 -> Divide/2

== matlab function adrc_main/Quad Dynamics1/Subsystem/z_dynamics/c_calc ==
  data: z input; c output; h input
function c = fcn(z, h)

if z > h/2
    c = 0;
elseif z < -h/2
    c = h;
else 
    c = h/2 - z;
end

== matlab function adrc_main/ADRC_yaw/TD1/fhan ==
  data: e input; u output; v2 input; r0 input; h0 input

function u = fhan(e, v2, r0, h0)

d = r0*h0^2;
a0 = h0*v2;
y = e + a0;

a1 = sqrt(d*(d + 8*abs(y)));
a2 = a0 + sign(y)*(a1 - d)/2;

sy = (sign(y + d) - sign(y - d))/2;
a = (a0 + y - a2)*sy + a2;

sa = (sign(a + d) - sign(a - d))/2;

u = -r0*(a/d - sign(a))*sa - r0*sign(a);

end

== matlab function adrc_main/ADRC_z/TD1/fhan ==
  data: e input; u output; v2 input; r0 input; h0 input

function u = fhan(e, v2, r0, h0)

d = r0*h0^2;
a0 = h0*v2;
y = e + a0;

a1 = sqrt(d*(d + 8*abs(y)));
a2 = a0 + sign(y)*(a1 - d)/2;

sy = (sign(y + d) - sign(y - d))/2;
a = (a0 + y - a2)*sy + a2;

sa = (sign(a + d) - sign(a - d))/2;

u = -r0*(a/d - sign(a))*sa - r0*sign(a);

end

== matlab function adrc_main/Quad Dynamics1/Subsystem/MATLAB Function ==
  data: U input; phi input; xdd output; theta input; psi input; Fx input; m input
function xdd = x_dynamics(U, phi, theta, psi, Fx, m)

T = U(1);
xdd = (T/m)*(cos(psi)*sin(theta)*cos(phi) ...
               + sin(psi)*sin(phi)) + Fx/m;

end

== matlab function adrc_main/Quad Dynamics1/Subsystem/MATLAB Function1 ==
  data: U input; ydd output; phi input; theta input; psi input; Fy input; m input
function ydd = y_dynamics(U, phi, theta, psi, Fy, m)

T = U(1);

ydd = (T/m)*(sin(psi)*sin(theta)*cos(phi) ...
               - cos(psi)*sin(phi)) + Fy/m;

end

== matlab function adrc_main/Quad Dynamics1/Subsystem/MATLAB Function2 ==
  data: phi input size=1; phidot output size=1; theta input size=1; p input size=1; q input size=1; r input size=1; U input; inertia_mx input; pdot output size=1
function [phidot, pdot] = roll_dynamics( ...
    phi, theta, p, q, r, U, inertia_mx)

Ix = inertia_mx(1);
Iy = inertia_mx(2);
Iz = inertia_mx(3);

tau_roll = U(2);

phidot = p + sin(phi)*tan(theta)*q ...
           + cos(phi)*tan(theta)*r;

pdot = (tau_roll + (Iy-Iz)*q*r)/Ix;

end

== matlab function adrc_main/Quad Dynamics1/Subsystem/MATLAB Function3 ==
  data: phi input size=1; thetadot output size=1; p input size=1; q input size=1; r input size=1; U input size=[4 1]; inertia_mx input size=[3 1]; qdot output size=1
function [thetadot, qdot] = pitch_dynamics( ...
    phi, p, q, r, U, inertia_mx)

Ix = inertia_mx(1);
Iy = inertia_mx(2);
Iz = inertia_mx(3);

tau_pitch = U(3);

thetadot = cos(phi)*q - sin(phi)*r;

qdot = (tau_pitch + (Iz-Ix)*p*r)/Iy;

end

== matlab function adrc_main/Quad Dynamics1/Subsystem/MATLAB Function4 ==
  data: phi input size=1; psidot output size=1; theta input size=1; p input size=1; q input size=1; r input size=1; U input; inertia_mx input; rdot output size=1
function [psidot, rdot] = yaw_dynamics( ...
    phi, theta, p, q, r, U, inertia_mx)

Ix = inertia_mx(1);
Iy = inertia_mx(2);
Iz = inertia_mx(3);

psidot = 0;
rdot = 0;

tau_yaw = U(4);

psidot = (sin(phi)*q + cos(phi)*r)/cos(theta);

rdot = (tau_yaw + (Ix-Iy)*p*q)/Iz;

end
